simulink model "Drag"  (R2026b)
settings: Solver=FixedStepAuto  StopTime=45  FixedStep=0.001
InitFcn:
  | altitudes = 0:3000:30000;
  | [T,a,P,densities] = atmosisa(altitudes);
values from neighbouring files (symbols this model uses):
  RCd_Clean = filloutliers(RCd_Clean,"pchip","movmedian",20)    [CdExtract.m]
  RCd_CleanAB = filloutliers(RCd_CleanAB,"pchip","movmedian",5)    [CdExtract.m]
undefined symbols (not defined in the file or in its folder): aerotech, o5500x, ps, Rmach_Clean, Rmach_CleanAB
libraries: aerolibatmos2 x2
settings Model: Creator=opore  LastModifiedBy=opore

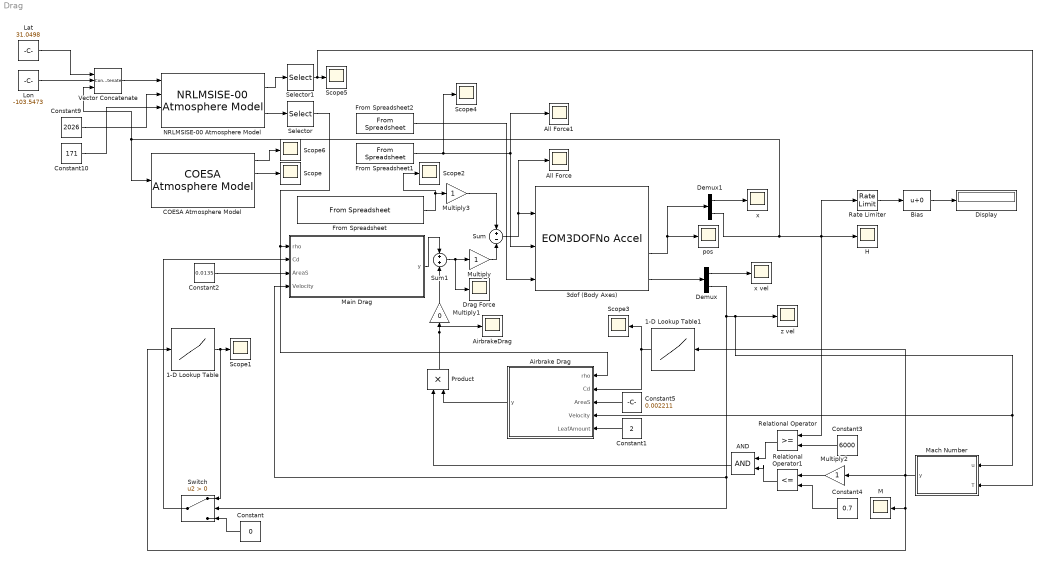
== system Drag ==
  1-D Lookup Table : Lookup_n-D  NumberOfTableDimensions=1  BreakpointsForDimension1=Rmach_Clean  Table=RCd_Clean  InternalRulePriority=Speed  RndMeth=Simplest
  1-D Lookup Table1 : Lookup_n-D  NumberOfTableDimensions=1  BreakpointsForDimension1=Rmach_CleanAB  Table=RCd_CleanAB  InternalRulePriority=Speed  RndMeth=Simplest
  3dof (Body Axes) : EOM3DOFNoAccel  mtype=Custom Variable  v_ini=0  theta_ini=-6*pi/180  alpha_ini=0.10471975512  pos_ini=[0 890]  mass=34  mass_e=24  mass_f=34  g=-9.81
  AND : Logic  IconShape=distinctive  AllPortsSameDT=off  OutDataTypeStr=boolean
  Airbrake Drag : MATLAB Function  TreatAsAtomicUnit=on
  AirbrakeDrag : Scope
      settings: ActiveDisplayYMinimum=-4.9578605067024037  ActiveDisplayYMaximum=43.749851110488294  DataLoggingVariableName=ScopeData12
  All Force : Scope
      settings: ActiveDisplayYMinimum=-5196.4604886640682  ActiveDisplayYMaximum=8206.2748778140485  DataLoggingVariableName=ScopeData4
  All Force1 : Scope
      settings: ActiveDisplayYMinimum=23.899625  ActiveDisplayYMaximum=36.123375  DataLoggingVariableName=ScopeData11
  Bias : Bias  SaturateOnIntegerOverflow=off
  COESA Atmosphere Model : aerolibatmos2/COESA Atmosphere Model  units=Metric (MKS)  spec=1976 COESA-extended U.S. Standard Atmosphere  model=Profile  profile_var=High temperature  profile_percent=1%  profile_alt=5 km (16404 ft)  envelope_var=High temperature  envelope_percent=1%  action=Warning
  Constant : Constant  Value=0
  Constant1 : Constant  Value=2
  Constant10 : Constant  Value=171
  Constant2 : Constant  Value=0.0135
  Constant3 : Constant  Value=6000
  Constant4 : Constant  Value=0.7
  Constant5 : Constant  Value=0.002211
  Constant9 : Constant  Value=2026
  Demux : Demux  Outputs=2
  Demux1 : Demux  Outputs=2
  Display : Display
  Drag Force : Scope
      settings: ActiveDisplayYMinimum=-2693.7398647025316  ActiveDisplayYMaximum=2774.4128105399077  DataLoggingVariableName=ScopeData3
  From Spreadsheet : FromSpreadsheet  FileName=/Users/opore/Desktop/Eat dog/ESM Daq/PLANAR_1/Plant_DEP/aerotech-o5500x-ps.xls  SheetName=aerotech-o5500x-ps  ExtrapolationBeforeFirstDataPoint=Ground value  ExtrapolationAfterLastDataPoint=Ground value
  From Spreadsheet1 : FromSpreadsheet  FileName=/Users/opore/Desktop/Eat dog/ESM Daq/PLANAR_1/Plant_DEP_A2/Macos/mass.xlsx  SheetName=mass  ExtrapolationBeforeFirstDataPoint=Ground value  ExtrapolationAfterLastDataPoint=Ground value
  From Spreadsheet2 : FromSpreadsheet  FileName=/Users/opore/Desktop/Eat dog/ESM Daq/PLANAR_1/Plant_DEP_A2/Macos/Rota.xlsx  SheetName=Rota  ExtrapolationBeforeFirstDataPoint=Ground value  ExtrapolationAfterLastDataPoint=Ground value
  H : Scope
      settings: ActiveDisplayYMinimum=-1880.9335198554345  ActiveDisplayYMaximum=12938.888819735039  DataLoggingVariableName=ScopeData6
  Lat : Constant  Value=31.0498
  Lon : Constant  Value=-103.5473
  M : Scope
      settings: ActiveDisplayYMinimum=-2.3417601116832509  ActiveDisplayYMaximum=3.5933295822030162  DataLoggingVariableName=ScopeData9
  Mach Number : MATLAB Function  TreatAsAtomicUnit=on
  Main Drag : MATLAB Function  TreatAsAtomicUnit=on
  Multiply : Gain
  Multiply1 : Gain  Gain=0
  Multiply2 : Gain
  Multiply3 : Gain
  NRLMSISE-00 Atmosphere Model : aerolibatmos2/NRLMSISE-00 Atmosphere Model  units=Metric (MKS)  lst_input=off  flux_ap_input=off  flags_input=Internal  flags=ones(1,23)  oxygen_in=off  action=Warning
  Product : Product
  Rate Limiter : RateLimiter  RisingSlewLimit=9999999999  FallingSlewLimit=0  SampleTimeMode=inherited
  Relational Operator : RelationalOperator  OutDataTypeStr=boolean  RndMeth=Simplest  InputSameDT=off
  Relational Operator1 : RelationalOperator  Operator=<=  OutDataTypeStr=boolean  RndMeth=Simplest  InputSameDT=off
  Scope{,1..6} (7 alike) : Scope
      Scope settings: ActiveDisplayYMinimum=257.45913595083135  ActiveDisplayYMaximum=358.063042902725  DataLoggingVariableName=ScopeData7
      Scope1 settings: ActiveDisplayYMinimum=0.142246068911414  ActiveDisplayYMaximum=2.2343271950039543  DataLoggingVariableName=ScopeData8
      Scope2 settings: ActiveDisplayYMinimum=-965.56124999999975  ActiveDisplayYMaximum=8690.05125  DataLoggingVariableName=ScopeData13
      Scope3 settings: ActiveDisplayYMinimum=-0.30993928651901759  ActiveDisplayYMaximum=2.11591791884692  DataLoggingVariableName=ScopeData10
      Scope4 settings: ActiveDisplayYMinimum=23.751625  ActiveDisplayYMaximum=35.975375  DataLoggingVariableName=ScopeData14
      Scope5 settings: ActiveDisplayYMinimum=220.05774557751454  ActiveDisplayYMaximum=300.81323362172  DataLoggingVariableName=ScopeData15
      Scope6 settings: ActiveDisplayYMinimum=209.4549696554767  ActiveDisplayYMaximum=290.46612105385378  DataLoggingVariableName=ScopeData16
  Selector : Selector  NumberOfDimensions=2  InputPortWidth=3  IndexOptions=Index vector (dialog),Index vector (dialog)  Indices=1,6  OutputSizes=1,1
  Selector1 : Selector  NumberOfDimensions=2  InputPortWidth=3  IndexOptions=Index vector (dialog),Index vector (dialog)  Indices=1,2  OutputSizes=1,1
  Sum : Sum  Inputs=+-
  Sum1 : Sum
  Switch : Switch  Criteria=u2 > Threshold  SaturateOnIntegerOverflow=off  InputSameDT=off
  Vector Concatenate : Concatenate  NumInputs=3  Mode=Multidimensional array  ConcatenateDimension=2
  pos : Scope
      settings: ActiveDisplayYMinimum=10609.328762883766  ActiveDisplayYMaximum=10634.804102146221
  x : Scope
      settings: ActiveDisplayYMinimum=-459.39156431028471  ActiveDisplayYMaximum=603.78982880719775  DataLoggingVariableName=ScopeData5
  x vel : Scope
      settings: ActiveDisplayYMinimum=-1.853501855089613  ActiveDisplayYMaximum=1.4042873984652722
  z vel : Scope
      settings: ActiveDisplayYMinimum=-974.10233461254859  ActiveDisplayYMaximum=1092.3737346711159  DataLoggingVariableName=ScopeData2
  wires:
  3dof (Body Axes)/3 -> pos/1, Demux1/1
  3dof (Body Axes)/4 -> Demux/1
  Demux/1 -> x vel/1
  Demux/2 -> Airbrake Drag/4(Velocity), Mach Number/1(u), z vel/1, Switch/2, Main Drag/4(Velocity)
  Sum/1 -> All Force/1, 3dof (Body Axes)/2
  Multiply/1 -> Sum/2
  Demux1/1 -> x/1
  1-D Lookup Table/1 -> Scope1/1, Switch/1
  Constant/1 -> Switch/3
  Constant2/1 -> Main Drag/3(AreaS)
  Switch/1 -> Main Drag/2(Cd)
  Constant5/1 -> Airbrake Drag/3(AreaS)
  Sum1/1 -> Drag Force/1, Multiply/1
  Main Drag/1(y) -> Sum1/1
  Constant3/1 -> Relational Operator/2
  Constant4/1 -> Relational Operator1/2
  Relational Operator/1 -> AND/1
  Relational Operator1/1 -> AND/2
  1-D Lookup Table1/1 -> Scope3/1, Airbrake Drag/2(Cd)
  Multiply1/1 -> Sum1/2
  AND/1 -> Product/1
  Airbrake Drag/1(y) -> Product/2
  Product/1 -> Multiply1/1, AirbrakeDrag/1
  Multiply2/1 -> Relational Operator1/1
  From Spreadsheet1/1 -> Scope4/1, All Force1/1, 3dof (Body Axes)/4
  From Spreadsheet2/1 -> 3dof (Body Axes)/6
  Mach Number/1(y) -> 1-D Lookup Table1/1, 1-D Lookup Table/1, M/1, Multiply2/1
  COESA Atmosphere Model/1 -> Scope6/1
  Constant1/1 -> Airbrake Drag/5(LeafAmount)
  From Spreadsheet/1 -> Scope2/1, Multiply3/1
  Multiply3/1 -> Sum/1
  Demux1/2 -> Vector Concatenate/3, COESA Atmosphere Model/1, Relational Operator/1, Rate Limiter/1, H/1
  COESA Atmosphere Model/2 -> Scope/1
  Rate Limiter/1 -> Bias/1
  Bias/1 -> Display/1
  Constant9/1 -> NRLMSISE-00 Atmosphere Model/2
  Constant10/1 -> NRLMSISE-00 Atmosphere Model/3
  Lat/1 -> Vector Concatenate/1
  Lon/1 -> Vector Concatenate/2
  Vector Concatenate/1 -> NRLMSISE-00 Atmosphere Model/1
  NRLMSISE-00 Atmosphere Model/2 -> Selector/1
  Selector/1 -> Airbrake Drag/1(rho), Main Drag/1(rho)
  NRLMSISE-00 Atmosphere Model/1 -> Selector1/1
  Selector1/1 -> Mach Number/2(T), Scope5/1

== matlab function Drag/Airbrake Drag ==
  data: y output; rho input; Cd input; AreaS input; Velocity input; LeafAmount input
function y = fcn(rho, Cd, AreaS, Velocity,LeafAmount)
    ForceDrag = LeafAmount*0.5*rho*Cd*AreaS*Velocity*abs(Velocity);
    y = ForceDrag;
end

== matlab function Drag/Main Drag ==
  data: y output; rho input; Cd input; AreaS input; Velocity input
function y = fcn(rho, Cd, AreaS, Velocity)
    ForceDrag = 0.5*rho*Cd*AreaS*Velocity*abs(Velocity);
    y = ForceDrag;
end

== matlab function Drag/Mach Number ==
  data: u input; y output; T input
function y = fcn(u,T)
rAir = 287.05;
specHeatAir = 1.4;
SoundC = sqrt(rAir*specHeatAir*T);
y = u/SoundC;
